simulink model "UnderwaterHideAndSeek"  (R2025b)
settings: Solver=FixedStepDiscrete  StartTime=0.0  StopTime=90.0  FixedStep=0.05  RelTol=1e-3
settings Model: Creator=ACER  LastModifiedBy=ACER

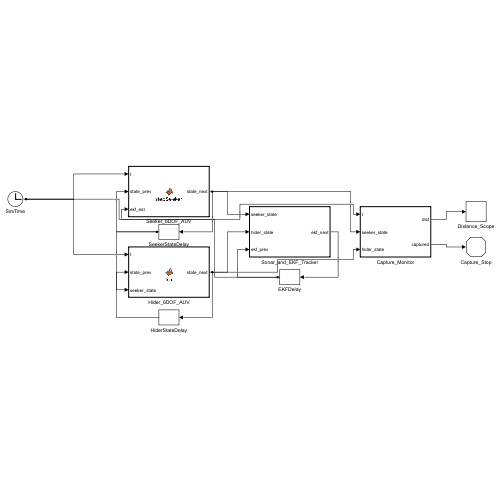
[thumbnail: Simulink's stored preview of the top-level diagram]
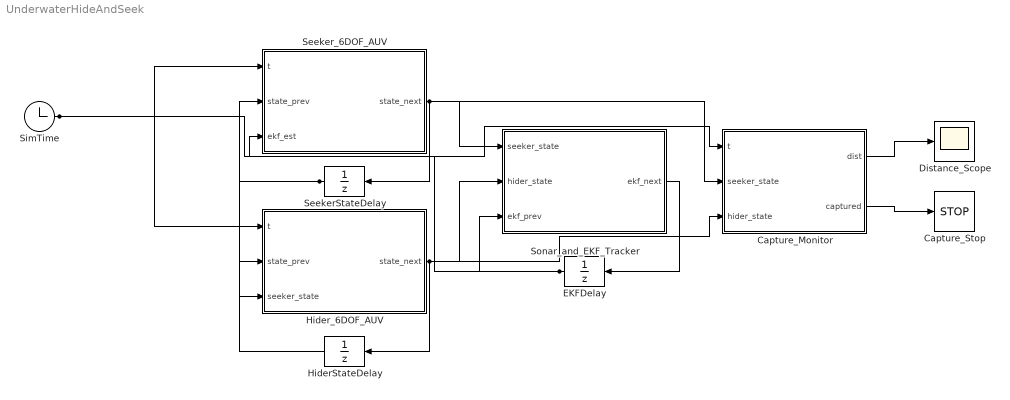
== system UnderwaterHideAndSeek ==
  Capture_Monitor : MATLAB Function  TreatAsAtomicUnit=on
  Capture_Stop : Stop
  Distance_Scope : Scope
  EKFDelay : UnitDelay  InitialCondition=[-10;-10;-14;0;0;0]  SampleTime=-1  HasFrameUpgradeWarning=on
  HiderStateDelay : UnitDelay  InitialCondition=[-12;-10;-14;0;0;0.5;0;0;0;0;0;0]  SampleTime=-1  HasFrameUpgradeWarning=on
  Hider_6DOF_AUV : MATLAB Function  TreatAsAtomicUnit=on
  SeekerStateDelay : UnitDelay  InitialCondition=[30;30;-10;0;0;-2.35;0;0;0;0;0;0]  SampleTime=-1  HasFrameUpgradeWarning=on
  Seeker_6DOF_AUV : MATLAB Function  TreatAsAtomicUnit=on
  SimTime : Clock
  Sonar_and_EKF_Tracker : MATLAB Function  TreatAsAtomicUnit=on
  wires:
  SimTime/1 -> Seeker_6DOF_AUV/1(t), Hider_6DOF_AUV/1(t), Capture_Monitor/1(t)
  SeekerStateDelay/1 -> Seeker_6DOF_AUV/2(state_prev), Hider_6DOF_AUV/3(seeker_state)
  EKFDelay/1 -> Seeker_6DOF_AUV/3(ekf_est), Sonar_and_EKF_Tracker/3(ekf_prev)
  Seeker_6DOF_AUV/1(state_next) -> SeekerStateDelay/1, Sonar_and_EKF_Tracker/1(seeker_state), Capture_Monitor/2(seeker_state)
  HiderStateDelay/1 -> Hider_6DOF_AUV/2(state_prev)
  Hider_6DOF_AUV/1(state_next) -> HiderStateDelay/1, Sonar_and_EKF_Tracker/2(hider_state), Capture_Monitor/3(hider_state)
  Sonar_and_EKF_Tracker/1(ekf_next) -> EKFDelay/1
  Capture_Monitor/1(dist) -> Distance_Scope/1
  Capture_Monitor/2(captured) -> Capture_Stop/1

== matlab function UnderwaterHideAndSeek/Hider_6DOF_AUV ==
  data: t input; state_next output; state_prev input; seeker_state input
function state_next = stepHider(t, state_prev, seeker_state)
% 6-DOF Hider Evasion AI + Fossen Hydrodynamics (dt = 0.05s)
dt = 0.05;
eta = state_prev(1:6); nu = state_prev(7:12);
p_h = eta(1:3); p_s = seeker_state(1:3);
away = p_h - p_s;
n = norm(away);
if n > 1e-3, dir = away / n; else, dir = [-1; -1; 0]; end
dir = dir + 0.45 * [-dir(2); dir(1); 0] * sin(0.35 * t);
v_des = (dir / max(1e-3, norm(dir))) * 1.45;
% Boundary repulsion
if p_h(1) < -50, v_des(1) = abs(v_des(1)); end
if p_h(1) >  50, v_des(1) = -abs(v_des(1)); end
if p_h(2) < -50, v_des(2) = abs(v_des(2)); end
if p_h(2) >  50, v_des(2) = -abs(v_des(2)); end
M = diag([17.0, 24.2, 26.07, 0.28, 0.28, 0.40]);
D = diag([4.03, 6.22, 5.18, 0.07, 0.07, 0.07]);
psi = eta(6);
R = [cos(psi) -sin(psi) 0; sin(psi) cos(psi) 0; 0 0 1];
v_world = R * nu(1:3);
f_body = R' * (30.0 * (v_des - v_world));
yaw_des = atan2(v_des(2), v_des(1));
e_yaw = atan2(sin(yaw_des - psi), cos(yaw_des - psi));
tau = [max(min(f_body, 35), -35); -8*eta(4)-2.5*nu(4); -8*eta(5)-2.5*nu(5); 10*e_yaw-3.5*nu(6)];
nu_dot = M \ (tau - D * nu);
nu_next = nu + dt * nu_dot;
eta_next = eta + dt * [R * nu_next(1:3); nu_next(4:6)];
eta_next(3) = max(min(eta_next(3), -1.0), -27.0);
state_next = [eta_next; nu_next];
end

== matlab function UnderwaterHideAndSeek/Seeker_6DOF_AUV ==
  data: t input; state_next output; state_prev input; ekf_est input
function state_next = stepSeeker(t, state_prev, ekf_est)
% 6-DOF Seeker Guidance + PID + Fossen Hydrodynamics (dt = 0.05s)
dt = 0.05;
eta = state_prev(1:6); nu = state_prev(7:12);
p = eta(1:3); target = ekf_est(1:3);
if t < 8.0
    v_des = [0; 0; 0];
else
    diff_t = target - p;
    n = norm(diff_t);
    if n > 1e-3, v_des = (diff_t / n) * 2.0; else, v_des = [0;0;0]; end
end
% Simple 6-DOF Fossen damping + proportional thrust
M = diag([17.0, 24.2, 26.07, 0.28, 0.28, 0.40]);
D = diag([4.03, 6.22, 5.18, 0.07, 0.07, 0.07]);
psi = eta(6);
R = [cos(psi) -sin(psi) 0; sin(psi) cos(psi) 0; 0 0 1];
v_world = R * nu(1:3);
f_world = 32.0 * (v_des - v_world);
f_body = R' * f_world;
yaw_des = atan2(target(2)-p(2), target(1)-p(1));
e_yaw = atan2(sin(yaw_des - psi), cos(yaw_des - psi));
tau = [max(min(f_body, 40), -40); -8*eta(4)-2.5*nu(4); -8*eta(5)-2.5*nu(5); 10*e_yaw-3.5*nu(6)];
nu_dot = M \ (tau - D * nu);
nu_next = nu + dt * nu_dot;
eta_next = eta + dt * [R * nu_next(1:3); nu_next(4:6)];
eta_next(3) = max(min(eta_next(3), -0.5), -28.0);
state_next = [eta_next; nu_next];
end

== matlab function UnderwaterHideAndSeek/Sonar_and_EKF_Tracker ==
  data: seeker_state input; ekf_next output; hider_state input; ekf_prev input
function ekf_next = stepEKF(seeker_state, hider_state, ekf_prev)
% Sonar Measurement + Alpha-Beta / EKF Target Tracker
dt = 0.05;
p_s = seeker_state(1:3); p_h = hider_state(1:3);
pos_pred = ekf_prev(1:3) + dt * ekf_prev(4:6);
vel_pred = 0.98 * ekf_prev(4:6);
dist = norm(p_h - p_s);
if dist <= 55.0
    alpha = 0.35; beta = 0.15;
    innov = p_h - pos_pred;
    pos_upd = pos_pred + alpha * innov;
    vel_upd = vel_pred + (beta / dt) * innov * 0.1;
    ekf_next = [pos_upd; vel_upd];
else
    ekf_next = [pos_pred; vel_pred];
end
end

== matlab function UnderwaterHideAndSeek/Capture_Monitor ==
  data: t input; dist output; seeker_state input; hider_state input; captured output
function [dist, captured] = monitorCapture(t, seeker_state, hider_state)
dist = norm(seeker_state(1:3) - hider_state(1:3));
captured = double(t >= 8.0 && dist <= 3.0);
end
